simulink model "Fig5_Falla_Desviacion_Ganancia"  (R2025b)
settings: Solver=ode4  StartTime=0.0  StopTime=0.6  FixedStep=2e-6  RelTol=1e-3
values from neighbouring files (symbols this model uses):
  x0 = [iL_ref; vc_ref]    [Parametros_Convertidor_Boost.m]
  xhat0 = [iL_ref; vc_ref]    [Parametros_Convertidor_Boost.m]
settings Model: Creator=ASUSTUF  LastModifiedBy=ASUSTUF

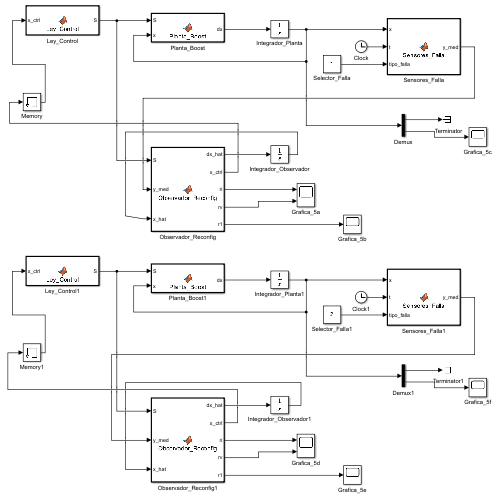
[thumbnail: Simulink's stored preview of the top-level diagram]
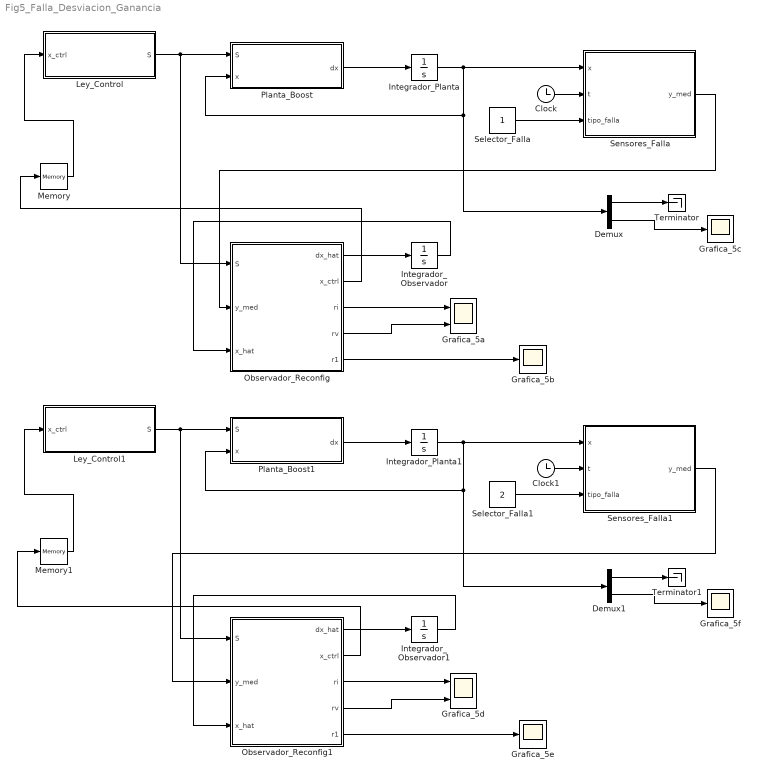
== system Fig5_Falla_Desviacion_Ganancia ==
  Clock : Clock
  Clock1 : Clock
  Demux : Demux  Outputs=2
  Demux1 : Demux  Outputs=2
  Grafica_5a : Scope  NumInputPorts=2
      settings: ActiveDisplayYMinimum=-3.983799605314891  ActiveDisplayYMaximum=5.128727366364437
  Grafica_5b : Scope
      settings: ActiveDisplayYMinimum=-0.35721716354630595  ActiveDisplayYMaximum=1.6268765437501749
  Grafica_5c : Scope
      settings: ActiveDisplayYMinimum=-1  ActiveDisplayYMaximum=1  DataLoggingVariableName=ScopeData2
  Grafica_5d : Scope  NumInputPorts=2
      settings: ActiveDisplayYMinimum=-388.24693022909986  ActiveDisplayYMaximum=-364.47010912175921  DataLoggingVariableName=ScopeData3
  Grafica_5e : Scope
      settings: ActiveDisplayYMinimum=-386.21135823386294  ActiveDisplayYMaximum=2136.8969921594071  DataLoggingVariableName=ScopeData4
  Grafica_5f : Scope
      settings: ActiveDisplayYMinimum=379.25309427002964  ActiveDisplayYMaximum=380.26684674592224  DataLoggingVariableName=ScopeData5
  Integrador_Observador : Integrator  InitialCondition=xhat0
  Integrador_Observador1 : Integrator  InitialCondition=xhat0
  Integrador_Planta : Integrator  InitialCondition=x0
  Integrador_Planta1 : Integrator  InitialCondition=x0
  Ley_Control : MATLAB Function  TreatAsAtomicUnit=on
  Ley_Control1 : MATLAB Function  TreatAsAtomicUnit=on
  Memory : Memory  InitialCondition=x0
  Memory1 : Memory  InitialCondition=x0
  Observador_Reconfig : MATLAB Function  TreatAsAtomicUnit=on
  Observador_Reconfig1 : MATLAB Function  TreatAsAtomicUnit=on
  Planta_Boost : MATLAB Function  TreatAsAtomicUnit=on
  Planta_Boost1 : MATLAB Function  TreatAsAtomicUnit=on
  Selector_Falla : Constant
  Selector_Falla1 : Constant  Value=2
  Sensores_Falla : MATLAB Function  TreatAsAtomicUnit=on
  Sensores_Falla1 : MATLAB Function  TreatAsAtomicUnit=on
  Terminator : Terminator
  Terminator1 : Terminator
  wires:
  Ley_Control/1(S) -> Observador_Reconfig/1(S), Planta_Boost/1(S)
  Planta_Boost/1(dx) -> Integrador_Planta/1
  Integrador_Planta/1 -> Demux/1, Planta_Boost/2(x), Sensores_Falla/1(x)
  Clock/1 -> Sensores_Falla/2(t)
  Selector_Falla/1 -> Sensores_Falla/3(tipo_falla)
  Sensores_Falla/1(y_med) -> Observador_Reconfig/2(y_med)
  Observador_Reconfig/1(dx_hat) -> Integrador_Observador/1
  Integrador_Observador/1 -> Observador_Reconfig/3(x_hat)
  Observador_Reconfig/3(ri) -> Grafica_5a/1
  Observador_Reconfig/4(rv) -> Grafica_5a/2
  Observador_Reconfig/5(r1) -> Grafica_5b/1
  Demux/2 -> Grafica_5c/1
  Demux/1 -> Terminator/1
  Observador_Reconfig/2(x_ctrl) -> Memory/1
  Memory/1 -> Ley_Control/1(x_ctrl)
  Integrador_Planta1/1 -> Demux1/1, Planta_Boost1/2(x), Sensores_Falla1/1(x)
  Demux1/2 -> Grafica_5f/1
  Clock1/1 -> Sensores_Falla1/2(t)
  Selector_Falla1/1 -> Sensores_Falla1/3(tipo_falla)
  Memory1/1 -> Ley_Control1/1(x_ctrl)
  Observador_Reconfig1/1(dx_hat) -> Integrador_Observador1/1
  Demux1/1 -> Terminator1/1
  Observador_Reconfig1/4(rv) -> Grafica_5d/2
  Observador_Reconfig1/5(r1) -> Grafica_5e/1
  Observador_Reconfig1/3(ri) -> Grafica_5d/1
  Observador_Reconfig1/2(x_ctrl) -> Memory1/1
  Ley_Control1/1(S) -> Observador_Reconfig1/1(S), Planta_Boost1/1(S)
  Integrador_Observador1/1 -> Observador_Reconfig1/3(x_hat)
  Sensores_Falla1/1(y_med) -> Observador_Reconfig1/2(y_med)
  Planta_Boost1/1(dx) -> Integrador_Planta1/1

== matlab function Fig5_Falla_Desviacion_Ganancia/Planta_Boost ==
  data: S input; dx output; x input
function dx = Planta_Boost(S, x)
Vin   = 190;
C0    = 0.00285;
L     = 0.005;
R     = 0.082;
Rload = 100;

A0 = [-R/L, -1/L; 1/C0, -1/(Rload*C0)];
A1 = [-R/L,  0;   0,    -1/(Rload*C0)];
B  = [1/L; 0];

if S == 0
    dx = A0 * x + B * Vin;
else
    dx = A1 * x + B * Vin;
end
end

== matlab function Fig5_Falla_Desviacion_Ganancia/Ley_Control ==
  data: x_ctrl input; S output
function S = Ley_Control(x_ctrl)
% Parámetros desde las ecuaciones del artículo
Vin   = 190;
C0    = 0.00285;
L     = 0.005;
R     = 0.082;
Rload = 100;

x_star = [7.6; 380];
P_lyap = [L, 0; 0, C0];

A0 = [-R/L, -1/L; 1/C0, -1/(Rload*C0)];
A1 = [-R/L,  0;   0,    -1/(Rload*C0)];
B  = [1/L; 0];

% Error de estado z = x - x*
z = x_ctrl - x_star;

% Derivadas de la función de Lyapunov V_dot para S=0 y S=1
V0_dot = 2 * z' * P_lyap * (A0 * x_ctrl + B * Vin);
V1_dot = 2 * z' * P_lyap * (A1 * x_ctrl + B * Vin);

% Regla de conmutación: elegir el modo con menor derivada
if V0_dot < V1_dot
    S = 0;
else
    S = 1;
end
end

== matlab function Fig5_Falla_Desviacion_Ganancia/Sensores_Falla ==
  data: x input; y_med output; t input; tipo_falla input
function y_med = Sensores_Falla(x, t, tipo_falla)
% x(1) = i_L, x(2) = v_c
% tipo_falla = 1 -> Desviación de ganancia en sensor de corriente (Fig. 5a, 5b, 5c)
% tipo_falla = 2 -> Desviación de ganancia en sensor de voltaje   (Fig. 5d, 5e, 5f)

y_med = x;

if t >= 0.2
    if tipo_falla == 1
        y_med(1) = 1.1 * x(1); % Aumento del 10% en la ganancia de corriente
    elseif tipo_falla == 2
        y_med(2) = 1.1 * x(2); % Aumento del 10% en la ganancia de voltaje
    end
end
end

== matlab function Fig5_Falla_Desviacion_Ganancia/Observador_Reconfig ==
  data: S input; dx_hat output; y_med input; x_hat input; x_ctrl output; ri output; rv output; r1 output
function [dx_hat, x_ctrl, ri, rv, r1] = Observador_Reconfig(S, y_med, x_hat)
Vin   = 190;
C0    = 0.00285;
L     = 0.005;
R     = 0.082;
Rload = 100;

x_star = [7.6; 380];
J_th   = 0.02;

H = [36.4677, -17.0967; 
     28.5219,  75.6359];

A0 = [-R/L, -1/L; 1/C0, -1/(Rload*C0)];
A1 = [-R/L,  0;   0,    -1/(Rload*C0)];
B  = [1/L; 0];

if S == 0
    A_s = A0;
else
    A_s = A1;
end

% 1. Generación de residuos (Ecuación 24)
y_hat = x_hat;
r = y_med - y_hat;
ri = r(1);
rv = r(2);
r1 = ri^2 + rv^2;

% 2. Detección de falla y Reconfiguración (Sección 5.2)
if r1 > J_th
    % Con alarma: se usa x_hat para el control y x* en el observador
    x_ctrl = x_hat;
    dx_hat = A_s * x_hat + B * Vin + H * (x_star - y_hat);
else
    % Sin alarma: operación normal con el valor medido y_med
    x_ctrl = y_med;
    dx_hat = A_s * x_hat + B * Vin + H * (y_med - y_hat);
end
end

== matlab function Fig5_Falla_Desviacion_Ganancia/Ley_Control1 ==
  data: x_ctrl input; S output
function S = Ley_Control(x_ctrl)
% Parámetros desde las ecuaciones del artículo
Vin   = 190;
C0    = 0.00285;
L     = 0.005;
R     = 0.082;
Rload = 100;

x_star = [7.6; 380];
P_lyap = [L, 0; 0, C0];

A0 = [-R/L, -1/L; 1/C0, -1/(Rload*C0)];
A1 = [-R/L,  0;   0,    -1/(Rload*C0)];
B  = [1/L; 0];

% Error de estado z = x - x*
z = x_ctrl - x_star;

% Derivadas de la función de Lyapunov V_dot para S=0 y S=1
V0_dot = 2 * z' * P_lyap * (A0 * x_ctrl + B * Vin);
V1_dot = 2 * z' * P_lyap * (A1 * x_ctrl + B * Vin);

% Regla de conmutación: elegir el modo con menor derivada
if V0_dot < V1_dot
    S = 0;
else
    S = 1;
end
end

== matlab function Fig5_Falla_Desviacion_Ganancia/Observador_Reconfig1 ==
  data: S input; dx_hat output; y_med input; x_hat input; x_ctrl output; ri output; rv output; r1 output
function [dx_hat, x_ctrl, ri, rv, r1] = Observador_Reconfig(S, y_med, x_hat)
Vin   = 190;
C0    = 0.00285;
L     = 0.005;
R     = 0.082;
Rload = 100;

x_star = [7.6; 380];
J_th   = 0.02;

H = [36.4677, -17.0967; 
     28.5219,  75.6359];

A0 = [-R/L, -1/L; 1/C0, -1/(Rload*C0)];
A1 = [-R/L,  0;   0,    -1/(Rload*C0)];
B  = [1/L; 0];

if S == 0
    A_s = A0;
else
    A_s = A1;
end

% 1. Generación de residuos (Ecuación 24)
y_hat = x_hat;
r = y_med - y_hat;
ri = r(1);
rv = r(2);
r1 = ri^2 + rv^2;

% 2. Detección de falla y Reconfiguración (Sección 5.2)
if r1 > J_th
    % Con alarma: se usa x_hat para el control y x* en el observador
    x_ctrl = x_hat;
    dx_hat = A_s * x_hat + B * Vin + H * (x_star - y_hat);
else
    % Sin alarma: operación normal con el valor medido y_med
    x_ctrl = y_med;
    dx_hat = A_s * x_hat + B * Vin + H * (y_med - y_hat);
end
end

== matlab function Fig5_Falla_Desviacion_Ganancia/Planta_Boost1 ==
  data: S input; dx output; x input
function dx = Planta_Boost(S, x)
Vin   = 190;
C0    = 0.00285;
L     = 0.005;
R     = 0.082;
Rload = 100;

A0 = [-R/L, -1/L; 1/C0, -1/(Rload*C0)];
A1 = [-R/L,  0;   0,    -1/(Rload*C0)];
B  = [1/L; 0];

if S == 0
    dx = A0 * x + B * Vin;
else
    dx = A1 * x + B * Vin;
end
end

== matlab function Fig5_Falla_Desviacion_Ganancia/Sensores_Falla1 ==
  data: x input; y_med output; t input; tipo_falla input
function y_med = Sensores_Falla(x, t, tipo_falla)
% x(1) = i_L, x(2) = v_c
% tipo_falla = 1 -> Desviación de ganancia en sensor de corriente (Fig. 5a, 5b, 5c)
% tipo_falla = 2 -> Desviación de ganancia en sensor de voltaje   (Fig. 5d, 5e, 5f)

y_med = x;

if t >= 0.2
    if tipo_falla == 1
        y_med(1) = 1.1 * x(1); % Aumento del 10% en la ganancia de corriente
    elseif tipo_falla == 2
        y_med(2) = 1.1 * x(2); % Aumento del 10% en la ganancia de voltaje
    end
end
end
